simulink model "FullFMS_2026_02_18_V0_3_9"  (R2025b)
settings: Solver=ode23tb  StartTime=0.0  StopTime=inf  MaxStep=0.1  RelTol=1e-2
PreLoadFcn:
  | load("BUS_CONFIG.mat")
libraries: opcualib x8
(part 2 of 4)

== matlab function FullFMS_2026_02_18_V0_3_9/MATLAB Function6 ==
  data: u1 input; A_94_Request output; u2 input; u3 input; u4 input; u5 input; u6 input; u7 input; u8 input; u9 input; u10 input; u11 input; u12 input; u13 input; u14 input; u15 input; u16 input; u17 input; u18 input; u19 input; u20 input; u21 input; u22 input; u23 input; u24 input; u25 input; u26 input; u27 input; u28 input; u29 input; u30 input; u31 input; u32 input; u33 input; u34 input; u35 input; u36 input; u37 input; u38 input; u39 input; u40 input; u41 input; u42 input; u43 input; u44 input; u45 input; u46 input; A_94_No_Cart output; A_94_Cart_Full output; A_94_CRoute_Out output; A_93_ProcCartID output; A_94_Cart_Stat output; A_94_Cart_Next output; A_94_Optic output; A_94_Count output; A_94_Pist_Bck output; A_94_Release_FB output; A_94_CRoute_In output; C_95_Initialization output; C_95_PD_Proc output; C_95_PD_Cart output; C_92_Profibus output; C_95_Start output; C_95_Cart2Del output; C_95_Del2Cart output; F_92_Claw_2_Cart output; F_92_Claw_2_Del output; F_92_Claw_Down output; F_92_Close_Claw output; F_93_Led_Start output; F_93_Led_Reset output; F_93_Led_Extra1 output; F_93_Led_Extra2 output; F_93_Panel_O4 output; F_93_Panel_O5 output; F_93_Panel_O6 output; F_93_Panel_O7 output; O_90_Part_Reserve output; O_90_Claw_Del output; O_90_Claw_Cart output; O_90_Claw_Reserve output; O_90_Claw_Low output; O_90_Claw_High output; O_90_Part_in_Claw output; O_91_Start output; O_91_Stop output; O_91_Key_Pos output; O_91_Reset output; O_91_Panel_I4 output; O_91_Panel_I5 output; O_91_Panel_I6 output; O_91_Panel_I7 output
function [A_94_Request, A_94_No_Cart, A_94_Cart_Full, A_94_CRoute_Out, ...
    A_93_ProcCartID, A_94_Cart_Stat, A_94_Cart_Next, A_94_Optic, A_94_Count, ...
    A_94_Pist_Bck, A_94_Release_FB, A_94_CRoute_In, ...
    C_95_Initialization, C_95_PD_Proc, C_95_PD_Cart, C_92_Profibus, ...
    C_95_Start, C_95_Cart2Del, C_95_Del2Cart, ...
    F_92_Claw_2_Cart, F_92_Claw_2_Del, F_92_Claw_Down, F_92_Close_Claw, ...
    F_93_Led_Start, F_93_Led_Reset, F_93_Led_Extra1, F_93_Led_Extra2, ...
    F_93_Panel_O4, F_93_Panel_O5, F_93_Panel_O6, F_93_Panel_O7, ...
    O_90_Part_Reserve, O_90_Claw_Del, O_90_Claw_Cart, O_90_Claw_Reserve, ...
    O_90_Claw_Low, O_90_Claw_High, O_90_Part_in_Claw, O_91_Start, O_91_Stop, ...
    O_91_Key_Pos, O_91_Reset, O_91_Panel_I4, O_91_Panel_I5, O_91_Panel_I6, ...
    O_91_Panel_I7] = ...
    fcn_HD2(u1, u2, u3, u4, u5, u6, u7, u8, u9, u10, u11, u12, ...
    u13, u14, u15, u16, u17, u18, u19, u20, u21, u22, u23, u24, u25, u26, ...
    u27, u28, u29, u30, u31, u32, u33, u34, u35, u36, u37, u38, u39, u40, ...
    u41, u42, u43, u44, u45, u46)

% Primeiro bloco - Asi (12 entradas: u1-u12)
A_94_Request = u1;
A_94_No_Cart = u2;
A_94_Cart_Full = u3;
A_94_CRoute_Out = u4;
A_93_ProcCartID = u5;
A_94_Cart_Stat = u6;
A_94_Cart_Next = u7;
A_94_Optic = u8;
A_94_Count = u9;
A_94_Pist_Bck = u10;
A_94_Release_FB = u11;
A_94_CRoute_In = u12;

% Segundo bloco - Control (7 entradas: u13-u19)
C_95_Initialization = u13;
C_95_PD_Proc = u14;
C_95_PD_Cart = u15;
C_92_Profibus = u16;
C_95_Start = u17;
C_95_Cart2Del = u18;
C_95_Del2Cart = u19;

% Terceiro bloco - Feedback (12 entradas: u20-u31)
F_92_Claw_2_Cart = u20;
F_92_Claw_2_Del = u21;
F_92_Claw_Down = u22;
F_92_Close_Claw = u23;
F_93_Led_Start = u24;
F_93_Led_Reset = u25;
F_93_Led_Extra1 = u26;
F_93_Led_Extra2 = u27;
F_93_Panel_O4 = u28;
F_93_Panel_O5 = u29;
F_93_Panel_O6 = u30;
F_93_Panel_O7 = u31;

% Quarto bloco - Sensors (15 entradas: u32-u46)
O_90_Part_Reserve = u32;
O_90_Claw_Del = u33;
O_90_Claw_Cart = u34;
O_90_Claw_Reserve = u35;
O_90_Claw_Low = u36;
O_90_Claw_High = u37;
O_90_Part_in_Claw = u38;
O_91_Start = u39;
O_91_Stop = u40;
O_91_Key_Pos = u41;
O_91_Reset = u42;
O_91_Panel_I4 = u43;
O_91_Panel_I5 = u44;
O_91_Panel_I6 = u45;
O_91_Panel_I7 = u46;

end

== matlab function FullFMS_2026_02_18_V0_3_9/MATLAB Function5 ==
  data: C_85_Initialization output; C_85_Part_Del output; C_85_Part_Mag output; C_86_Mag_Parts output; C_87_RQ_MParts output; C_82_Profibus output; C_83_RQ_Parts output; C_85_Start output; C_85_Single output; C_85_Continuous output; C_85_Counted output; F_82_Pist_Adv output; F_82_Suction_On output; F_82_Suction_Off output; F_82_Arm_2_Del output; F_82_Arm_2_Mag output; F_83_Led_Start output; F_83_Led_Reset output; F_83_Led_Extra1 output; F_83_Led_Extra2 output; F_83_Panel_O4 output; F_83_Panel_O5 output; F_83_Panel_O6 output; F_83_Panel_O7 output; O_80_Mag_Full output; O_80_Pist_Back output; O_80_Pist_Fwd output; O_80_Part_Stuck output; O_80_Arm_Mag output; O_80_Arm_Del output; O_80_Mag_Empty output; O_81_Start output; O_81_Stop output; O_81_Key_Pos output; O_81_Reset output; O_81_Panel_I4 output; O_81_Panel_I5 output; O_81_Panel_I6 output; O_81_Panel_I7 output; u1 input; u2 input; u3 input; u4 input; u5 input; u6 input; u7 input; u8 input; u9 input; u10 input; u11 input; u12 input; u13 input; u14 input; u15 input; u16 input; u17 input; u18 input; u19 input; u20 input; u21 input; u22 input; u23 input; u24 input; u25 input; u26 input; u27 input; u28 input; u29 input; u30 input; u31 input; u32 input; u33 input; u34 input; u35 input; u36 input; u37 input; u38 input; u39 input
function [C_85_Initialization, C_85_Part_Del, C_85_Part_Mag, C_86_Mag_Parts, ...
    C_87_RQ_MParts, C_82_Profibus, C_83_RQ_Parts, C_85_Start, C_85_Single, ...
    C_85_Continuous, C_85_Counted, ...
    F_82_Pist_Adv, F_82_Suction_On, F_82_Suction_Off, F_82_Arm_2_Del, ...
    F_82_Arm_2_Mag, F_83_Led_Start, F_83_Led_Reset, F_83_Led_Extra1, ...
    F_83_Led_Extra2, F_83_Panel_O4, F_83_Panel_O5, F_83_Panel_O6, F_83_Panel_O7, ...
    O_80_Mag_Full, O_80_Pist_Back, O_80_Pist_Fwd, O_80_Part_Stuck, ...
    O_80_Arm_Mag, O_80_Arm_Del, O_80_Mag_Empty, O_81_Start, O_81_Stop, ...
    O_81_Key_Pos, O_81_Reset, O_81_Panel_I4, O_81_Panel_I5, O_81_Panel_I6, ...
    O_81_Panel_I7] = ...
    fcn_DIST(u1, u2, u3, u4, u5, u6, u7, u8, u9, u10, u11, ...
    u12, u13, u14, u15, u16, u17, u18, u19, u20, u21, u22, u23, u24, u25, ...
    u26, u27, u28, u29, u30, u31, u32, u33, u34, u35, u36, u37, u38, u39)

% Primeiro bloco - Controls (11 entradas: u1-u11)
C_85_Initialization = u1;
C_85_Part_Del = u2;
C_85_Part_Mag = u3;
C_86_Mag_Parts = u4;
C_87_RQ_MParts = u5;
C_82_Profibus = u6;
C_83_RQ_Parts = u7;
C_85_Start = u8;
C_85_Single = u9;
C_85_Continuous = u10;
C_85_Counted = u11;

% Segundo bloco - Feedbacks (13 entradas: u12-u24)
F_82_Pist_Adv = u12;
F_82_Suction_On = u13;
F_82_Suction_Off = u14;
F_82_Arm_2_Del = u15;
F_82_Arm_2_Mag = u16;
F_83_Led_Start = u17;
F_83_Led_Reset = u18;
F_83_Led_Extra1 = u19;
F_83_Led_Extra2 = u20;
F_83_Panel_O4 = u21;
F_83_Panel_O5 = u22;
F_83_Panel_O6 = u23;
F_83_Panel_O7 = u24;

% Terceiro bloco - Sensors (15 entradas: u25-u39)
O_80_Mag_Full = u25;
O_80_Pist_Back = u26;
O_80_Pist_Fwd = u27;
O_80_Part_Stuck = u28;
O_80_Arm_Mag = u29;
O_80_Arm_Del = u30;
O_80_Mag_Empty = u31;
O_81_Start = u32;
O_81_Stop = u33;
O_81_Key_Pos = u34;
O_81_Reset = u35;
O_81_Panel_I4 = u36;
O_81_Panel_I5 = u37;
O_81_Panel_I6 = u38;
O_81_Panel_I7 = u39;

end

== matlab function FullFMS_2026_02_18_V0_3_9/MATLAB Function4 ==
  data: u1 input; A_74_Request output; u2 input; u3 input; u4 input; u5 input; u6 input; u7 input; u8 input; u9 input; u10 input; u11 input; u12 input; u13 input; u14 input; u15 input; u16 input; u17 input; u18 input; u19 input; u20 input; u21 input; u22 input; u23 input; u24 input; u25 input; u26 input; u27 input; u28 input; u29 input; u30 input; u31 input; u32 input; u33 input; u34 input; u35 input; u36 input; u37 input; u38 input; u39 input; u40 input; u41 input; u42 input; u43 input; u44 input; u45 input; u46 input; u47 input; u48 input; u49 input; u50 input; u51 input; u52 input; u53 input; A_74_No_Cart output; A_74_Cart_Full output; A_74_CRoute_Out output; A_74_CRoute_In80 output; A_73_TestCartID output; A_74_Cart_Stat output; A_74_Cart_Next output; A_74_Optic output; A_74_Count output; A_74_Pist_Bck output; A_74_Release_FB output; A_74_CRoute_In output; C_75_Initialization output; C_75_ID_Delivery1 output; C_75_ID_Delivery2 output; C_75_Part_Del output; C_75_RQ_Part_Del output; C_75_RQ_Wrong output; C_75_Identified80 output; C_75_Requested80 output; C_72_Profibus output; C_75_RQ_Delivery1 output; C_75_RQ_Delivery2 output; C_75_Identified output; C_75_Requested output; F_72_Elev_Down output; F_72_Elev_Up output; F_72_Eject_Part output; F_72_Air_On output; F_73_Led_Start output; F_73_Led_Reset output; F_73_Led_Extra1 output; F_73_Led_Extra2 output; F_73_Panel_O4 output; F_73_Panel_O5 output; F_73_Panel_O6 output; F_73_Panel_O7 output; O_70_SInductive output; O_70_SPart output; O_70_SStation output; O_70_SPart_Height output; O_70_Elev_High output; O_70_Elev_Low output; O_70_Pist_Back output; O_71_Start output; O_71_Stop output; O_71_Key_Pos output; O_71_Reset output; O_71_Panel_I4 output; O_71_Panel_I5 output; O_71_Panel_I6 output; O_71_Panel_I7 output
function [A_74_Request, A_74_No_Cart, A_74_Cart_Full, A_74_CRoute_Out, ...
    A_74_CRoute_In80, A_73_TestCartID, A_74_Cart_Stat, A_74_Cart_Next, ...
    A_74_Optic, A_74_Count, A_74_Pist_Bck, A_74_Release_FB, A_74_CRoute_In, ...
    C_75_Initialization, C_75_ID_Delivery1, C_75_ID_Delivery2, C_75_Part_Del, ...
    C_75_RQ_Part_Del, C_75_RQ_Wrong, C_75_Identified80, C_75_Requested80, ...
    C_72_Profibus, C_75_RQ_Delivery1, C_75_RQ_Delivery2, C_75_Identified, ...
    C_75_Requested, ...
    F_72_Elev_Down, F_72_Elev_Up, F_72_Eject_Part, F_72_Air_On, ...
    F_73_Led_Start, F_73_Led_Reset, F_73_Led_Extra1, F_73_Led_Extra2, ...
    F_73_Panel_O4, F_73_Panel_O5, F_73_Panel_O6, F_73_Panel_O7, ...
    O_70_SInductive, O_70_SPart, O_70_SStation, O_70_SPart_Height, ...
    O_70_Elev_High, O_70_Elev_Low, O_70_Pist_Back, O_71_Start, O_71_Stop, ...
    O_71_Key_Pos, O_71_Reset, O_71_Panel_I4, O_71_Panel_I5, O_71_Panel_I6, ...
    O_71_Panel_I7] = ...
    fcn_TEST(u1, u2, u3, u4, u5, u6, u7, u8, u9, u10, u11, u12, u13, ...
    u14, u15, u16, u17, u18, u19, u20, u21, u22, u23, u24, u25, u26, u27, ...
    u28, u29, u30, u31, u32, u33, u34, u35, u36, u37, u38, u39, u40, u41, ...
    u42, u43, u44, u45, u46, u47, u48, u49, u50, u51, u52, u53)

% Primeiro bloco - Asi (13 entradas: u1-u13)
A_74_Request = u1;
A_74_No_Cart = u2;
A_74_Cart_Full = u3;
A_74_CRoute_Out = u4;
A_74_CRoute_In80 = u5;
A_73_TestCartID = u6;
A_74_Cart_Stat = u7;
A_74_Cart_Next = u8;
A_74_Optic = u9;
A_74_Count = u10;
A_74_Pist_Bck = u11;
A_74_Release_FB = u12;
A_74_CRoute_In = u13;

% Segundo bloco - Control (13 entradas: u14-u26)
C_75_Initialization = u14;
C_75_ID_Delivery1 = u15;
C_75_ID_Delivery2 = u16;
C_75_Part_Del = u17;
C_75_RQ_Part_Del = u18;
C_75_RQ_Wrong = u19;
C_75_Identified80 = u20;
C_75_Requested80 = u21;
C_72_Profibus = u22;
C_75_RQ_Delivery1 = u23;
C_75_RQ_Delivery2 = u24;
C_75_Identified = u25;
C_75_Requested = u26;

% Terceiro bloco - Feedback (12 entradas: u27-u38)
F_72_Elev_Down = u27;
F_72_Elev_Up = u28;
F_72_Eject_Part = u29;
F_72_Air_On = u30;
F_73_Led_Start = u31;
F_73_Led_Reset = u32;
F_73_Led_Extra1 = u33;
F_73_Led_Extra2 = u34;
F_73_Panel_O4 = u35;
F_73_Panel_O5 = u36;
F_73_Panel_O6 = u37;
F_73_Panel_O7 = u38;

% Quarto bloco - Sensors (15 entradas: u39-u53)
O_70_SInductive = u39;
O_70_SPart = u40;
O_70_SStation = u41;
O_70_SPart_Height = u42;
O_70_Elev_High = u43;
O_70_Elev_Low = u44;
O_70_Pist_Back = u45;
O_71_Start = u46;
O_71_Stop = u47;
O_71_Key_Pos = u48;
O_71_Reset = u49;
O_71_Panel_I4 = u50;
O_71_Panel_I5 = u51;
O_71_Panel_I6 = u52;
O_71_Panel_I7 = u53;

end

== matlab function FullFMS_2026_02_18_V0_3_9/MATLAB Function7 ==
  data: u1 input; C_105_Initialization output; u2 input; u3 input; u4 input; u5 input; u6 input; u7 input; u8 input; u9 input; u10 input; u11 input; u12 input; u13 input; u14 input; u15 input; u16 input; u17 input; u18 input; u19 input; u20 input; u21 input; u22 input; u23 input; u24 input; u25 input; u26 input; u27 input; u28 input; u29 input; u30 input; u31 input; u32 input; u33 input; u34 input; u35 input; u36 input; u37 input; u38 input; u39 input; C_105_Part_ready output; C_105_Test_Ok output; C_105_Test_Fail output; C_102_Profibus output; C_103_RQ_Turns output; C_105_Start output; C_105_Test output; C_105_TestDrill output; C_105_Rotation output; F_102_Drill_On output; F_102_RT_On output; F_102_Drill_Down output; F_102_Drill_Up output; F_102_Drill_Pin output; F_102_Test_Pin output; F_103_Led_Start output; F_103_Led_Reset output; F_103_Led_Extra1 output; F_103_Led_Extra2 output; F_103_Panel_O4 output; F_103_Panel_O5 output; F_103_Panel_O6 output; F_103_Panel_O7 output; O_100_PInit_Pos output; O_100_PDrill_Pos output; O_100_PTest_Pos output; O_100_SDrill_High output; O_100_SDrill_Low output; O_100_RT_Sensor output; O_100_PTest_Ok output; O_101_Start output; O_101_Stop output; O_101_Key_Pos output; O_101_Reset output; O_101_Panel_I4 output; O_101_Panel_I5 output; O_101_Panel_I6 output; O_101_Panel_I7 output
function [C_105_Initialization, C_105_Part_ready, C_105_Test_Ok, ...
    C_105_Test_Fail, C_102_Profibus, C_103_RQ_Turns, C_105_Start, ...
    C_105_Test, C_105_TestDrill, C_105_Rotation, ...
    F_102_Drill_On, F_102_RT_On, F_102_Drill_Down, F_102_Drill_Up, ...
    F_102_Drill_Pin, F_102_Test_Pin, F_103_Led_Start, F_103_Led_Reset, ...
    F_103_Led_Extra1, F_103_Led_Extra2, F_103_Panel_O4, F_103_Panel_O5, ...
    F_103_Panel_O6, F_103_Panel_O7, ...
    O_100_PInit_Pos, O_100_PDrill_Pos, O_100_PTest_Pos, O_100_SDrill_High, ...
    O_100_SDrill_Low, O_100_RT_Sensor, O_100_PTest_Ok, O_101_Start, ...
    O_101_Stop, O_101_Key_Pos, O_101_Reset, O_101_Panel_I4, O_101_Panel_I5, ...
    O_101_Panel_I6, O_101_Panel_I7] = ...
    fcn_PROC(u1, u2, u3, u4, u5, u6, u7, u8, u9, u10, ...
    u11, u12, u13, u14, u15, u16, u17, u18, u19, u20, u21, u22, u23, u24, ...
    u25, u26, u27, u28, u29, u30, u31, u32, u33, u34, u35, u36, u37, u38, u39)

% Primeiro bloco - Control (10 entradas: u1-u10)
C_105_Initialization = u1;
C_105_Part_ready = u2;
C_105_Test_Ok = u3;
C_105_Test_Fail = u4;
C_102_Profibus = u5;
C_103_RQ_Turns = u6;
C_105_Start = u7;
C_105_Test = u8;
C_105_TestDrill = u9;
C_105_Rotation = u10;

% Segundo bloco - Feedback (14 entradas: u11-u24)
F_102_Drill_On   = u11;
F_102_RT_On      = u12;
F_102_Drill_Down = u13;
F_102_Drill_Up   = u14;
F_102_Drill_Pin  = u15;
F_102_Test_Pin   = u16;
F_103_Led_Start  = u17;
F_103_Led_Reset  = u18;
F_103_Led_Extra1 = u19;
F_103_Led_Extra2 = u20;
F_103_Panel_O4   = u21;
F_103_Panel_O5   = u22;
F_103_Panel_O6   = u23;
F_103_Panel_O7   = u24;

% Terceiro bloco - Sensors (15 entradas: u25-u39)
O_100_PInit_Pos   = u25;
O_100_PDrill_Pos  = u26;
O_100_PTest_Pos   = u27;
O_100_SDrill_High = u28;
O_100_SDrill_Low  = u29;
O_100_RT_Sensor   = u30;
O_100_PTest_Ok    = u31;
O_101_Start       = u32;
O_101_Stop        = u33;
O_101_Key_Pos     = u34;
O_101_Reset       = u35;
O_101_Panel_I4    = u36;
O_101_Panel_I5    = u37;
O_101_Panel_I6    = u38;
O_101_Panel_I7    = u39;

end
